simulink model "hmfc_fic1_simscape"  (R2026a)
settings: Solver=ode15s  StopTime=c.duration  MaxStep=0.005  RelTol=1e-9  AbsTol=1e-10
InitFcn:
  | assignin(get_param(bdroot,'ModelWorkspace'),'c',hmfc_parameters());
model workspace (MAT data in the model file):
  c.l1 = 0.6
  c.l2 = 0.5
  c.m1 = 2
  c.m2 = 1.5
  c.lc1 = 0.3
  c.lc2 = 0.25
  c.I1 = 0.06
  c.I2 = 0.03125
  c.g = 9.81
  c.kp = 25
  c.kv = 10
  c.fd = 10
  c.surfaceAngle = 0
  c.n = [0; 1]
  c.T = [1; 0]
  c.p0 = [0.6; 0.4]
  c.initialVelocity = 0
  c.q2Min = 1.2217304764
  c.q2Max = 2.00712863979
  c.minSinQ2 = 0.906307787037
  c.xMin = -0.04
  c.xMax = 0.16
  c.q0 = [-0.167329366792; 1.72136459957]
  c.dq0 = [0; 0]
  c.targetX = 0.08
  c.setpoint = [0.68; 0.4]
  c.duration = 6
  c.outputStep = 0.002
  kf = 0
  mode = 0
values from neighbouring files (symbols this model uses):
  c = hmfc_parameters()    [build_hmfc_simscape.m]    (also in fic1_simscape_simulation.m)
undefined symbols (not defined in the file or in its folder): X, Y, Z
libraries: sm_lib x12, nesl_utility x10, simulink x1
settings Model: Creator=zichen24  LastModifiedBy=zichen24
settings SolverCC: AlgebraicLoopSolver=LineSearch
settings ExplorerConfigSet: SimMechanicsOpenEditorOnUpdate=off

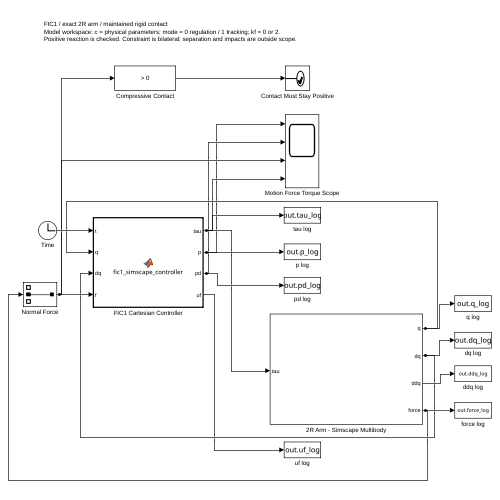
[thumbnail: Simulink's stored preview of the top-level diagram]
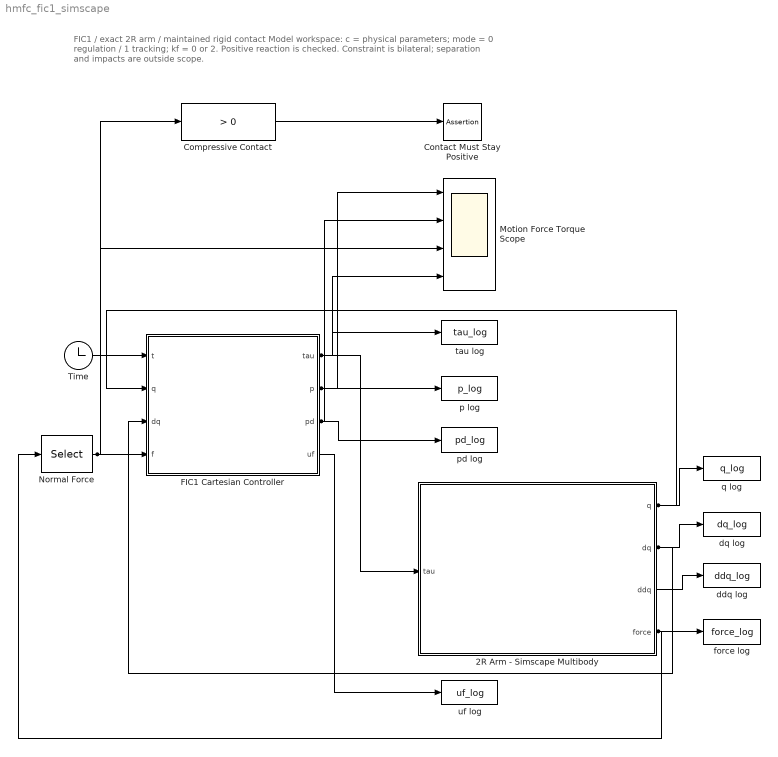
== system hmfc_fic1_simscape ==
  note: FIC1 / exact 2R arm / maintained rigid contact
      | Model workspace: c = physical parameters; mode = 0 regulation / 1 tracking; kf = 0 or 2.
      | Positive reaction is checked. Constraint is bilateral; separation and impacts are outside scope.
  2R Arm - Simscape Multibody : Subsystem
  Compressive Contact : simulink/Logic and Bit Operations/Compare To Constant  relop=>  const=0  OutDataTypeStr=boolean
  Contact Must Stay Positive : Assertion
  FIC1 Cartesian Controller : MATLAB Function  TreatAsAtomicUnit=on
  Motion Force Torque Scope : Scope  NumInputPorts=4
  Normal Force : Selector  InputPortWidth=3  IndexOptions=Index vector (dialog)  Indices=2  OutputSizes=1
  Time : Clock
  ddq log : ToWorkspace  VariableName=ddq_log  SaveFormat=Timeseries  SampleTime=-1
  dq log : ToWorkspace  VariableName=dq_log  SaveFormat=Timeseries  SampleTime=-1
  force log : ToWorkspace  VariableName=force_log  SaveFormat=Timeseries  SampleTime=-1
  p log : ToWorkspace  VariableName=p_log  SaveFormat=Timeseries  SampleTime=-1
  pd log : ToWorkspace  VariableName=pd_log  SaveFormat=Timeseries  SampleTime=-1
  q log : ToWorkspace  VariableName=q_log  SaveFormat=Timeseries  SampleTime=-1
  tau log : ToWorkspace  VariableName=tau_log  SaveFormat=Timeseries  SampleTime=-1
  uf log : ToWorkspace  VariableName=uf_log  SaveFormat=Timeseries  SampleTime=-1
  wires:
  2R Arm - Simscape Multibody/3(ddq) -> ddq log/1
  2R Arm - Simscape Multibody/2(dq) -> dq log/1, FIC1 Cartesian Controller/3(dq)
  FIC1 Cartesian Controller/4(uf) -> uf log/1
  2R Arm - Simscape Multibody/4(force) -> force log/1, Normal Force/1
  FIC1 Cartesian Controller/3(pd) -> Motion Force Torque Scope/2, pd log/1
  FIC1 Cartesian Controller/1(tau) -> Motion Force Torque Scope/4, tau log/1, 2R Arm - Simscape Multibody/1(tau)
  Compressive Contact/1 -> Contact Must Stay Positive/1
  Normal Force/1 -> Compressive Contact/1, FIC1 Cartesian Controller/4(f), Motion Force Torque Scope/3
  2R Arm - Simscape Multibody/1(q) -> q log/1, FIC1 Cartesian Controller/2(q)
  FIC1 Cartesian Controller/2(p) -> Motion Force Torque Scope/1, p log/1
  Time/1 -> FIC1 Cartesian Controller/1(t)

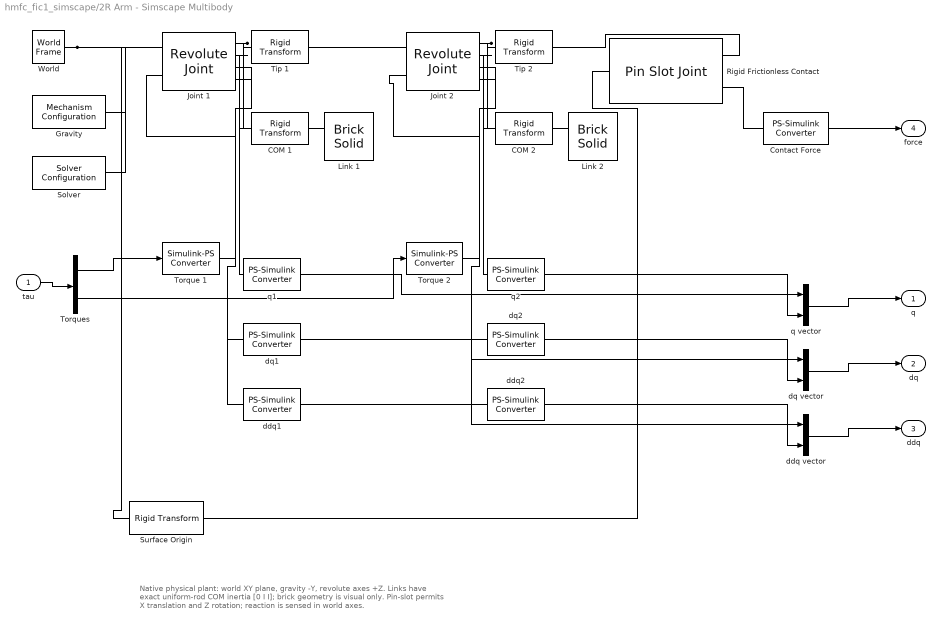
== system hmfc_fic1_simscape/2R Arm - Simscape Multibody ==
  note: Native physical plant: world XY plane, gravity -Y, revolute axes +Z.
      | Links have exact uniform-rod COM inertia [0 I I]; brick geometry is visual only.
      | Pin-slot permits X translation and Z rotation; reaction is sensed in world axes.
  tau : Inport
  COM 1 : sm_lib/Frames and Transforms/Rigid Transform  RotationMethod=None  FollAlignAxisA=+X  BaseAlignAxisA=+Y  FollAlignAxisB=+Y  BaseAlignAxisB=+Z  RotationStandardAxis=+Z  RotationAngle=0  RotationAngleUnits=deg  RotationArbitraryAxis=[0 0 1]  RotationSequenceAxes=FollowerAxes  RotationSequence=XYX  RotationSequenceAngles=[0 0 0]  RotationSequenceAnglesUnits=deg  RotationMatrix=[1 0 0;0 1 0;0 0 1]  Quaternion=[1 0 0 0]  TranslationMethod=Cartesian  TranslationCartesianOffset=[c.lc1 0 0]  TranslationCartesianOffsetUnits=m  TranslationStandardAxis=+Z  TranslationStandardOffset=0  TranslationStandardOffsetUnits=m  TranslationROffset=0  TranslationROffsetUnits=m  TranslationThetaOffset=0  TranslationThetaOffsetUnits=deg  TranslationZOffset=0  TranslationZOffsetUnits=m
  COM 2 : sm_lib/Frames and Transforms/Rigid Transform  RotationMethod=None  FollAlignAxisA=+X  BaseAlignAxisA=+Y  FollAlignAxisB=+Y  BaseAlignAxisB=+Z  RotationStandardAxis=+Z  RotationAngle=0  RotationAngleUnits=deg  RotationArbitraryAxis=[0 0 1]  RotationSequenceAxes=FollowerAxes  RotationSequence=XYX  RotationSequenceAngles=[0 0 0]  RotationSequenceAnglesUnits=deg  RotationMatrix=[1 0 0;0 1 0;0 0 1]  Quaternion=[1 0 0 0]  TranslationMethod=Cartesian  TranslationCartesianOffset=[c.lc2 0 0]  TranslationCartesianOffsetUnits=m  TranslationStandardAxis=+Z  TranslationStandardOffset=0  TranslationStandardOffsetUnits=m  TranslationROffset=0  TranslationROffsetUnits=m  TranslationThetaOffset=0  TranslationThetaOffsetUnits=deg  TranslationZOffset=0  TranslationZOffsetUnits=m
  Contact Force : nesl_utility/PS-Simulink Converter  PhysicalDomain=network_engine_domain  SubClassName=ps_output  LeftPortType=input  RightPortType=output  PseudoPeriodic=off  Frequencies=[]  VectorFormat=inherit  Unit=N  AffineConversion=off
  Gravity : sm_lib/Utilities/Mechanism Configuration  UniformGravity=Constant  GravityVector=[0 -c.g 0]  GravityVectorUnits=m/s^2  LinearizationDelta=0.001  JointModeTransitionNonlinearIterations=2
  Joint 1 : sm_lib/Joints/Revolute Joint  JointMode=Normal  CompositeWrenchDir=FollowerOnBase  CompositeWrenchFrame=BaseFrame  SenseConstraintForce=off  SenseConstraintTorque=off  SenseTotalForce=off  SenseTotalTorque=off  PositionTargetSpecify=on  PositionTargetPriority=High  PositionTargetValue=c.q0(1)  PositionTargetValueUnits=rad  VelocityTargetSpecify=on  VelocityTargetPriority=High  VelocityTargetValue=c.dq0(1)  VelocityTargetValueUnits=rad/s  EquilibriumPosition=0  EquilibriumPositionUnits=deg  SpringStiffness=0  SpringStiffnessUnits=N*m/deg  DampingCoefficient=0  DampingCoefficientUnits=N*m/(deg/s)  LowerLimitSpecify=off  LowerLimitBound=-90  LowerLimitBoundUnits=deg  LowerLimitStiffness=1e4  LowerLimitStiffnessUnits=N*m/deg  LowerLimitDamping=10  LowerLimitDampingUnits=N*m/(deg/s)  LowerLimitTransitionRegionWidth=0.1  LowerLimitTransitionRegionWidthUnits=deg  UpperLimitSpecify=off  UpperLimitBound=90  UpperLimitBoundUnits=deg  UpperLimitStiffness=1e4  UpperLimitStiffnessUnits=N*m/deg  UpperLimitDamping=10  UpperLimitDampingUnits=N*m/(deg/s)  UpperLimitTransitionRegionWidth=0.1  UpperLimitTransitionRegionWidthUnits=deg  TorqueActuationMode=InputTorque  MotionActuationMode=ComputedMotion  SensePosition=on  SenseVelocity=on  SenseAcceleration=on  SenseTorqueForce=off  SenseLowerLimitTorqueForce=off  SenseUpperLimitTorqueForce=off
  Joint 2 : sm_lib/Joints/Revolute Joint  JointMode=Normal  CompositeWrenchDir=FollowerOnBase  CompositeWrenchFrame=BaseFrame  SenseConstraintForce=off  SenseConstraintTorque=off  SenseTotalForce=off  SenseTotalTorque=off  PositionTargetSpecify=on  PositionTargetPriority=High  PositionTargetValue=c.q0(2)  PositionTargetValueUnits=rad  VelocityTargetSpecify=on  VelocityTargetPriority=High  VelocityTargetValue=c.dq0(2)  VelocityTargetValueUnits=rad/s  EquilibriumPosition=0  EquilibriumPositionUnits=deg  SpringStiffness=0  SpringStiffnessUnits=N*m/deg  DampingCoefficient=0  DampingCoefficientUnits=N*m/(deg/s)  LowerLimitSpecify=off  LowerLimitBound=-90  LowerLimitBoundUnits=deg  LowerLimitStiffness=1e4  LowerLimitStiffnessUnits=N*m/deg  LowerLimitDamping=10  LowerLimitDampingUnits=N*m/(deg/s)  LowerLimitTransitionRegionWidth=0.1  LowerLimitTransitionRegionWidthUnits=deg  UpperLimitSpecify=off  UpperLimitBound=90  UpperLimitBoundUnits=deg  UpperLimitStiffness=1e4  UpperLimitStiffnessUnits=N*m/deg  UpperLimitDamping=10  UpperLimitDampingUnits=N*m/(deg/s)  UpperLimitTransitionRegionWidth=0.1  UpperLimitTransitionRegionWidthUnits=deg  TorqueActuationMode=InputTorque  MotionActuationMode=ComputedMotion  SensePosition=on  SenseVelocity=on  SenseAcceleration=on  SenseTorqueForce=off  SenseLowerLimitTorqueForce=off  SenseUpperLimitTorqueForce=off
  Link 1 : sm_lib/Body Elements/Brick Solid  BrickDimensions=[c.l1 0.025 0.025]  BrickDimensionsUnits=m  ExportEntireGeometry=off  InertiaType=Custom  BasedOnType=Density  Density=1000  DensityUnits=kg/m^3  Mass=c.m1  MassUnits=kg  CenterOfMass=[0 0 0]  CenterOfMassUnits=m  MomentsOfInertia=[0 c.I1 c.I1]  MomentsOfInertiaUnits=kg*m^2  ProductsOfInertia=[0 0 0]  ProductsOfInertiaUnits=kg*m^2  GraphicType=FromGeometry  MarkerShape=Sphere  MarkerSize=10  GraphicVisPropType=SimpleVisualProperties  GraphicDiffuseColor=[0.1 0.4 0.8]  GraphicOpacity=1  GraphicSpecularColor=[0.5 0.5 0.5 1.0]  GraphicAmbientColor=[0.15 0.15 0.15 1.0]  GraphicEmissiveColor=[0.0 0.0 0.0 1.0]  GraphicShininess=75  DoExposeReferenceFrame=on  SerializedFrames=<Frames/>
  Link 2 : sm_lib/Body Elements/Brick Solid  BrickDimensions=[c.l2 0.025 0.025]  BrickDimensionsUnits=m  ExportEntireGeometry=off  InertiaType=Custom  BasedOnType=Density  Density=1000  DensityUnits=kg/m^3  Mass=c.m2  MassUnits=kg  CenterOfMass=[0 0 0]  CenterOfMassUnits=m  MomentsOfInertia=[0 c.I2 c.I2]  MomentsOfInertiaUnits=kg*m^2  ProductsOfInertia=[0 0 0]  ProductsOfInertiaUnits=kg*m^2  GraphicType=FromGeometry  MarkerShape=Sphere  MarkerSize=10  GraphicVisPropType=SimpleVisualProperties  GraphicDiffuseColor=[0.9 0.45 0.1]  GraphicOpacity=1  GraphicSpecularColor=[0.5 0.5 0.5 1.0]  GraphicAmbientColor=[0.15 0.15 0.15 1.0]  GraphicEmissiveColor=[0.0 0.0 0.0 1.0]  GraphicShininess=75  DoExposeReferenceFrame=on  SerializedFrames=<Frames/>
  Rigid Frictionless Contact : sm_lib/Joints/Pin Slot Joint  JointMode=Normal  CompositeWrenchDir=BaseOnFollower  CompositeWrenchFrame=BaseFrame  SenseConstraintForce=on  SenseConstraintTorque=off  SenseTotalForce=off  SenseTotalTorque=off  PxPositionTargetSpecify=off  PxPositionTargetPriority=High  PxPositionTargetValue=0  PxPositionTargetValueUnits=m  PxVelocityTargetSpecify=off  PxVelocityTargetPriority=High  PxVelocityTargetValue=0  PxVelocityTargetValueUnits=m/s  PxEquilibriumPosition=0  PxEquilibriumPositionUnits=m  PxSpringStiffness=0  PxSpringStiffnessUnits=N/m  PxDampingCoefficient=0  PxDampingCoefficientUnits=N/(m/s)  PxLowerLimitSpecify=off  PxLowerLimitBound=-1  PxLowerLimitBoundUnits=m  PxLowerLimitStiffness=1e6  PxLowerLimitStiffnessUnits=N/m  PxLowerLimitDamping=1e3  PxLowerLimitDampingUnits=N/(m/s)  PxLowerLimitTransitionRegionWidth=1e-4  PxLowerLimitTransitionRegionWidthUnits=m  PxUpperLimitSpecify=off  PxUpperLimitBound=1  PxUpperLimitBoundUnits=m  PxUpperLimitStiffness=1e6  PxUpperLimitStiffnessUnits=N/m  PxUpperLimitDamping=1e3  PxUpperLimitDampingUnits=N/(m/s)  PxUpperLimitTransitionRegionWidth=1e-4  PxUpperLimitTransitionRegionWidthUnits=m  PxTorqueActuationMode=NoTorque  PxMotionActuationMode=ComputedMotion  PxSensePosition=off  PxSenseVelocity=off  PxSenseAcceleration=off  PxSenseTorqueForce=off  PxSenseLowerLimitTorqueForce=off  PxSenseUpperLimitTorqueForce=off  RzPositionTargetSpecify=off  RzPositionTargetPriority=High  RzPositionTargetValue=0  RzPositionTargetValueUnits=deg  RzVelocityTargetSpecify=off  RzVelocityTargetPriority=High  RzVelocityTargetValue=0  RzVelocityTargetValueUnits=deg/s  RzEquilibriumPosition=0  RzEquilibriumPositionUnits=deg  RzSpringStiffness=0  RzSpringStiffnessUnits=N*m/deg  RzDampingCoefficient=0  RzDampingCoefficientUnits=N*m/(deg/s)  RzLowerLimitSpecify=off  RzLowerLimitBound=-90  RzLowerLimitBoundUnits=deg  RzLowerLimitStiffness=1e4  RzLowerLimitStiffnessUnits=N*m/deg  RzLowerLimitDamping=10  RzLowerLimitDampingUnits=N*m/(deg/s)  RzLowerLimitTransitionRegionWidth=0.1  RzLowerLimitTransitionRegionWidthUnits=deg  RzUpperLimitSpecify=off  RzUpperLimitBound=90  RzUpperLimitBoundUnits=deg  RzUpperLimitStiffness=1e4  RzUpperLimitStiffnessUnits=N*m/deg  RzUpperLimitDamping=10  RzUpperLimitDampingUnits=N*m/(deg/s)  RzUpperLimitTransitionRegionWidth=0.1  RzUpperLimitTransitionRegionWidthUnits=deg  RzTorqueActuationMode=NoTorque  RzMotionActuationMode=ComputedMotion  RzSensePosition=off  RzSenseVelocity=off  RzSenseAcceleration=off  RzSenseTorqueForce=off  RzSenseLowerLimitTorqueForce=off  RzSenseUpperLimitTorqueForce=off
  Solver : nesl_utility/Solver Configuration  PhysicalDomain=network_engine_domain  SubClassName=solver  LeftPortType=input  RightPortType=generic  Tones=[]  Harmonics=[]  SimulateNoise=off  Profile=off  UseLocalSampling=off  EnableSwitchedLinearOptims=on  FrequencyDomain=off  UseCCode=off  RelTol=0.001  AbsTol=0.001  MinStep=1e-09  ToWorkspace=off  RevertToSquareIcSolve=off  NumHomotopyIterations=100  PhasorMode=off  PhasorModeNumHarmonics=1  ConsistencySolver=NEWTON_XTOL_AFTER_FTOL  CanonicalOrdering=CANONICAL  OptimizeIntermediates=OPTIMIZED  IndexReductionMethod=DerivativeReplacement  DoDC=off  ResidualTolerance=1e-09  ConsistencyTolSource=GLOBAL  ConsistencyAbsTol=0.001  ConsistencyRelTol=0.001  ConsistencyTolFactor=0.001  UseLocalSolver=off  LocalSolverChoice=NE_BACKWARD_EULER_ADVANCER  ResolveIndetEquations=on  FunctionEvalNumThread=1  LocalSolverSampleTime=0.001  DoFixedCost=off  MaxNonlinIter=3  MaxModeIter=2  ComputeImpulses=off  ImpulseIterations=2  LinearAlgebra=auto  LinearAlgebraNumThread=0  EquationFormulation=NE_TIME_EF  DelaysMemoryBudget=1024  AutomaticFiltering=on  FilteringTimeConstant=0.001  PartitionStorageMethod=AS_NEEDED  PartitionMemoryBudget=1024  PartitionMethod=ROBUST  MultibodyUseLocalSolver=off  MultibodyLocalSolverChoice=ODE1  MultibodyLocalSolverSampleTime=0.001
  Surface Origin : sm_lib/Frames and Transforms/Rigid Transform  RotationMethod=None  FollAlignAxisA=+X  BaseAlignAxisA=+Y  FollAlignAxisB=+Y  BaseAlignAxisB=+Z  RotationStandardAxis=+Z  RotationAngle=0  RotationAngleUnits=deg  RotationArbitraryAxis=[0 0 1]  RotationSequenceAxes=FollowerAxes  RotationSequence=XYX  RotationSequenceAngles=[0 0 0]  RotationSequenceAnglesUnits=deg  RotationMatrix=[1 0 0;0 1 0;0 0 1]  Quaternion=[1 0 0 0]  TranslationMethod=Cartesian  TranslationCartesianOffset=[c.p0(1) c.p0(2) 0]  TranslationCartesianOffsetUnits=m  TranslationStandardAxis=+Z  TranslationStandardOffset=0  TranslationStandardOffsetUnits=m  TranslationROffset=0  TranslationROffsetUnits=m  TranslationThetaOffset=0  TranslationThetaOffsetUnits=deg  TranslationZOffset=0  TranslationZOffsetUnits=m
  Tip 1 : sm_lib/Frames and Transforms/Rigid Transform  RotationMethod=None  FollAlignAxisA=+X  BaseAlignAxisA=+Y  FollAlignAxisB=+Y  BaseAlignAxisB=+Z  RotationStandardAxis=+Z  RotationAngle=0  RotationAngleUnits=deg  RotationArbitraryAxis=[0 0 1]  RotationSequenceAxes=FollowerAxes  RotationSequence=XYX  RotationSequenceAngles=[0 0 0]  RotationSequenceAnglesUnits=deg  RotationMatrix=[1 0 0;0 1 0;0 0 1]  Quaternion=[1 0 0 0]  TranslationMethod=Cartesian  TranslationCartesianOffset=[c.l1 0 0]  TranslationCartesianOffsetUnits=m  TranslationStandardAxis=+Z  TranslationStandardOffset=0  TranslationStandardOffsetUnits=m  TranslationROffset=0  TranslationROffsetUnits=m  TranslationThetaOffset=0  TranslationThetaOffsetUnits=deg  TranslationZOffset=0  TranslationZOffsetUnits=m
  Tip 2 : sm_lib/Frames and Transforms/Rigid Transform  RotationMethod=None  FollAlignAxisA=+X  BaseAlignAxisA=+Y  FollAlignAxisB=+Y  BaseAlignAxisB=+Z  RotationStandardAxis=+Z  RotationAngle=0  RotationAngleUnits=deg  RotationArbitraryAxis=[0 0 1]  RotationSequenceAxes=FollowerAxes  RotationSequence=XYX  RotationSequenceAngles=[0 0 0]  RotationSequenceAnglesUnits=deg  RotationMatrix=[1 0 0;0 1 0;0 0 1]  Quaternion=[1 0 0 0]  TranslationMethod=Cartesian  TranslationCartesianOffset=[c.l2 0 0]  TranslationCartesianOffsetUnits=m  TranslationStandardAxis=+Z  TranslationStandardOffset=0  TranslationStandardOffsetUnits=m  TranslationROffset=0  TranslationROffsetUnits=m  TranslationThetaOffset=0  TranslationThetaOffsetUnits=deg  TranslationZOffset=0  TranslationZOffsetUnits=m
  Torque 1 : nesl_utility/Simulink-PS Converter  PhysicalDomain=network_engine_domain  SubClassName=ps_input  LeftPortType=input  RightPortType=output  PseudoPeriodic=off  Frequencies=[]  NoiseDistribution=none  NoiseParameters=[]  Unit=N*m  AffineConversion=off  FilteringAndDerivatives=provide  SimscapeFilterOrder=1  InputFilterTimeConstant=0.001  UdotUserProvided=0
  Torque 2 : nesl_utility/Simulink-PS Converter  PhysicalDomain=network_engine_domain  SubClassName=ps_input  LeftPortType=input  RightPortType=output  PseudoPeriodic=off  Frequencies=[]  NoiseDistribution=none  NoiseParameters=[]  Unit=N*m  AffineConversion=off  FilteringAndDerivatives=provide  SimscapeFilterOrder=1  InputFilterTimeConstant=0.001  UdotUserProvided=0
  Torques : Demux  Outputs=2
  World : sm_lib/Frames and Transforms/World Frame
  ddq vector : Mux  Inputs=2
  ddq1 : nesl_utility/PS-Simulink Converter  PhysicalDomain=network_engine_domain  SubClassName=ps_output  LeftPortType=input  RightPortType=output  PseudoPeriodic=off  Frequencies=[]  VectorFormat=inherit  Unit=rad/s^2  AffineConversion=off
  ddq2 : nesl_utility/PS-Simulink Converter  PhysicalDomain=network_engine_domain  SubClassName=ps_output  LeftPortType=input  RightPortType=output  PseudoPeriodic=off  Frequencies=[]  VectorFormat=inherit  Unit=rad/s^2  AffineConversion=off
  dq vector : Mux  Inputs=2
  dq1 : nesl_utility/PS-Simulink Converter  PhysicalDomain=network_engine_domain  SubClassName=ps_output  LeftPortType=input  RightPortType=output  PseudoPeriodic=off  Frequencies=[]  VectorFormat=inherit  Unit=rad/s  AffineConversion=off
  dq2 : nesl_utility/PS-Simulink Converter  PhysicalDomain=network_engine_domain  SubClassName=ps_output  LeftPortType=input  RightPortType=output  PseudoPeriodic=off  Frequencies=[]  VectorFormat=inherit  Unit=rad/s  AffineConversion=off
  q vector : Mux  Inputs=2
  q1 : nesl_utility/PS-Simulink Converter  PhysicalDomain=network_engine_domain  SubClassName=ps_output  LeftPortType=input  RightPortType=output  PseudoPeriodic=off  Frequencies=[]  VectorFormat=inherit  Unit=rad  AffineConversion=off
  q2 : nesl_utility/PS-Simulink Converter  PhysicalDomain=network_engine_domain  SubClassName=ps_output  LeftPortType=input  RightPortType=output  PseudoPeriodic=off  Frequencies=[]  VectorFormat=inherit  Unit=rad  AffineConversion=off
  q : Outport
  dq : Outport  Port=2
  ddq : Outport  Port=3
  force : Outport  Port=4
  wires:
  tau/1 -> Torques/1
  Torques/1 -> Torque 1/1
  Torques/2 -> Torque 2/1
  q1/1 -> q vector/1
  q2/1 -> q vector/2
  q vector/1 -> q/1
  dq1/1 -> dq vector/1
  dq2/1 -> dq vector/2
  dq vector/1 -> dq/1
  ddq1/1 -> ddq vector/1
  ddq2/1 -> ddq vector/2
  ddq vector/1 -> ddq/1
  Contact Force/1 -> force/1
  connections:
  Gravity/RConn1 -- World/RConn1 -- Solver/RConn1 -- Joint 1/LConn1 -- Surface Origin/LConn1
  COM 1/LConn1 -- Joint 1/RConn1 -- Tip 1/LConn1
  COM 1/RConn1 -- Link 1/RConn1
  Torque 1/RConn1 -- Joint 1/LConn2
  Joint 1/RConn2 -- q1/LConn1
  Joint 1/RConn3 -- dq1/LConn1
  Joint 1/RConn4 -- ddq1/LConn1
  COM 2/LConn1 -- Joint 2/RConn1 -- Tip 2/LConn1
  COM 2/RConn1 -- Link 2/RConn1
  Torque 2/RConn1 -- Joint 2/LConn2
  Joint 2/RConn2 -- q2/LConn1
  Joint 2/RConn3 -- dq2/LConn1
  Joint 2/RConn4 -- ddq2/LConn1
  Tip 1/RConn1 -- Joint 2/LConn1
  Surface Origin/RConn1 -- Rigid Frictionless Contact/LConn1
  Tip 2/RConn1 -- Rigid Frictionless Contact/RConn1
  Rigid Frictionless Contact/RConn2 -- Contact Force/LConn1

== matlab function hmfc_fic1_simscape/FIC1 Cartesian Controller ==
  data: t input; tau output; q input; dq input; f input; p output; pd output; uf output; c parameter; mode parameter; kf parameter
function [tau,p,pd,uf] = fic1_simscape_controller(t,q,dq,f,c, mode, kf)
%#codegen
%FIC1_SIMSCAPE_CONTROLLER Cartesian FIC1; q,dq,f come from Multibody sensors.
% This function is embedded in the generated model's MATLAB Function block.
% c, mode (0 regulation, 1 tracking), kf are model-workspace parameters.
s1=sin(q(1)); c1=cos(q(1));
s12=sin(q(1)+q(2)); c12=cos(q(1)+q(2));
p=[c.l1*c1+c.l2*c12;c.l1*s1+c.l2*s12];
J=[-c.l1*s1-c.l2*s12,-c.l2*s12;c.l1*c1+c.l2*c12,c.l2*c12];
v=J*dq;
if mode==0
    pd=c.p0+c.T*c.targetX;
    dpd=zeros(2,1); ddpd=zeros(2,1);
else
    pd=c.p0+c.T*(0.08+0.045*sin(0.8*t)+0.02*cos(1.3*t));
    dpd=c.T*(0.045*0.8*cos(0.8*t)-0.02*1.3*sin(1.3*t));
    ddpd=c.T*(-0.045*0.8^2*sin(0.8*t)-0.02*1.3^2*cos(1.3*t));
end
A=c.I1+c.m1*c.lc1^2+c.m2*c.l1^2;
B=c.m2*c.l1*c.lc2; D=c.I2+c.m2*c.lc2^2;
M=[A+D+2*B*cos(q(2)),D+B*cos(q(2));D+B*cos(q(2)),D];
b=B*sin(q(2));
C=[-b*dq(2),-b*(dq(1)+dq(2));b*dq(1),0];
G=[(c.m1*c.lc1+c.m2*c.l1)*c.g*c1+c.m2*c.lc2*c.g*c12;c.m2*c.lc2*c.g*c12];
dJdq=-[c.l1*c1*dq(1)^2+c.l2*c12*(dq(1)+dq(2))^2; ...
    c.l1*s1*dq(1)^2+c.l2*s12*(dq(1)+dq(2))^2];
up=ddpd+c.kv*(dpd-v)+c.kp*(pd-p);
uf=c.fd+kf*(c.fd-f);
% tau = J'*(eta + Lambda*up - n*uf), evaluated without explicit inverse.
tau=C*dq+G+M*(J\(up-dJdq))-J'*c.n*uf;
end
